simulink model "psm_sv_ekf_bemf_ctrl"  (R2026a)
settings: Solver=ode23tb  StopTime=simlength  FixedStep=tc  MaxStep=tc
values from neighbouring files (symbols this model uses):
  A1_tilde_ekf = [-Rs_norm/Lalpha_norm 0 0 0 0 0; 0 -Rs_norm/Lalpha_norm 0 0 0 0;      0 0 0 0 0 0; 0 0 0 0 0 0;      0 0 0 0 0 1; 0 0 0 0 0 0]    [kalman_psm.m]
  A2_tilde_ekf = [0 0 0 1/Lbeta_norm 0 0; 0 0 -1/Lbeta_norm 0 0 0;      0 0 0 -1 0 0; 0 0 1 0 0 0;     0 0 0 0 0 0; 0 0 0 0 0 0]    [kalman_psm.m]
  A3_tilde_ekf = [0 0 0 0 0 0; 0 0 0 0 0 -1/Lbeta_norm;      0 0 0 0 0 0; 0 0 0 0 0 1;     0 0 0 0 0 0; 0 0 0 0 0 0]    [kalman_psm.m]
  A4_tilde_ekf = [0 0 0 0 0 1/Lalpha_norm; 0 0 0 0 0 0;      0 0 0 0 0 -1; 0 0 0 0 0 0;     0 0 0 0 0 0; 0 0 0 0 0 0]    [kalman_psm.m]
  Bd_ekf = B_tilde_ekf*ts_inv    [kalman_psm.m]
  C_ekf = [1 0 0 0 0 0; 0 1 0 0 0 0]    [kalman_psm.m]
  CTRPIFF_CLIP_RELEASE = 0.001    [init_model.m]
  dead_time_INV = 3e-6    (= 3e-06)    [init_model.m]
  fPWM_INV = fPWM_AFE    (= 5000)    [init_model.m]
  g0_10Hz = fcut_10Hz_flt * ts_afe * 2*pi    (= 0.0125663706144)    [init_model.m]
  g0_1Hz = fcut_1Hz_flt * ts_afe * 2*pi    (= 0.00125663706144)    [init_model.m]
  g1_10Hz = 1 - g0_10Hz    (= 0.987433629386)    [init_model.m]
  g1_1Hz = 1 - g0_1Hz    (= 0.998743362939)    [init_model.m]
  id_lim = 0.35    [init_model.m]
  inv_m_scale = motorc_m_scale    [init_model.m]
  iq_lim = 1.4    [init_model.m]
  kg = Kobs(1)    [init_model.m]
  ki_align = 0.1    [init_model.m]
  ki_i = 18    [init_model.m]
  ki_w = 8    [init_model.m]
  kp_align = 0.6    [init_model.m]
  kp_i = 0.25    [init_model.m]
  kp_w = 2    [init_model.m]
  kw = Kobs(2)    [init_model.m]
  lim_down_align = -0.2    [init_model.m]
  lim_up_align = 0.2    [init_model.m]
  number_of_modules = 1    [init_model.m]
  omega_m_sim = omega_m_bez    [init_model.m]
  Qkalman = ts_inv * [Rs_norm/Lalpha_norm 0 0 0 0 0; 0 Rs_norm/Lbeta_norm 0 0 0 0;      0 0 1 0 0 0;     0 0 0 1 0 0;     0 0 0 0 1 0;     0 0 0 0 0 1]    [kalman_psm.m]
  Rkalman = [ts_inv 0; 0 ts_inv]    [kalman_psm.m]
  simlength = 2    [init_model.m]
  tc = ts_afe/100    (= 2e-06)    [init_model.m]
  time_gain_afe_module_1 = 1.0    (= 1)    [init_model.m]
  time_gain_inv_module_2 = 1.0    (= 1)    [init_model.m]
  time_start_motor_control = 0.025    [init_model.m]
  ts_inv = 1/fPWM_INV    (= 0.0002)    [init_model.m]
undefined symbols (not defined in the file or in its folder): ibez, La, Lb, Ld_norm, Lq_norm, magnitude, omega_bez, omega_m_bez, psi_bez, psi_m, rpm_base, rpm_bez, Rs, tau_bez, torque_base, ubez
libraries: fl_lib x24, nesl_utility x11, cstblocks_lti x2, single_phase_pwm_modulator x1, threephase_inductor_lib x1, simple_flexible_shaft x1, permanent_magnet_synchronous_machine x1
(part 1 of 2)
settings Model: SimulationMode=accelerator  Creator=dbagn  LastModifiedBy=ltnbda
settings SolverCC: NumberNewtonIterations=3.0  ZeroCrossControl=DisableAll  SolverResetMethod=Robust
settings SFSimCC: CustomCodeUndefinedFunction=ThrowError  DefaultCustomCodeDeterministicFunctions=All
settings SFSimCC: SimCustomHeaderCode=|
  | #include "rpi.h"
  | #include "mavgflt.h"
  | #include "mavgflt_simulink.h"
  | #include "mavgflts.h"
  | #include "mavgflts_simulink.h"
  | #include "dsmavgflt.h"
  | #include "dsmavgflt_simulink.h"
  | #include "bemf_obsv.h"
  | #include "bemf_obsv_simulink.h"
  | #include "bemf_obsv_load_est.h"
  | #include "bemf_obsv_load_est_simulink.h"
  | #include "dqvector_pi.h"
  | #include "dqvector_pi_simulink.h"
  | #include "sv_pwm_simulink.h"
  | #include "sv_pwm.h"
  | #include "first_harmonic_tracker.h"
  | #include "first_harmonic_tracker_simulink.h"
  | #include "dqpll_thyr.h"
  | #include "dqpll_thyr_simulink.h"
  | #include "dqpll_grid.h"
  | #include "dqpll_grid_simulink.h"
settings SFSimCC: SimUserSources=|
  | "rpi.c"
  | "mavgflt_simulink.c"
  | "mavgflt.c"
  | "mavgflts_simulink.c"
  | "mavgflts.c"
  | "dsmavgflt_simulink.c"
  | "dsmavgflt.c"
  | "bemf_obsv_simulink.c"
  | "bemf_obsv.c"
  | "bemf_obsv_load_est_simulink.c"
  | "bemf_obsv_load_est.c"
  | "dqvector_pi.c"
  | "dqvector_pi_simulink.c"
  | "sv_pwm_simulink.c"
  | "sv_pwm.c"
  | "first_harmonic_tracker_simulink.c"
  | "first_harmonic_tracker.c"
  | "dqpll_thyr_simulink.c"
  | "dqpll_thyr.c"
  | "dqpll_grid_simulink.c"
  | "dqpll_grid.c"
settings SFSimCC: SimUserIncludeDirs=|
  | include
  | src
settings SimscapeCC: SimscapeNominalValues="[{\"value\":\"1\",\"unit\":\"A\"},{\"value\":\"1\",\"unit\":\"bar\"},{\"value\":\"1\",\"unit\":\"cm^2\"},{\"value\":\"1\",\"unit\":\"cm^3/s\"},{\"value\":\"1\",\"unit\":\"kJ/kg\"},{\"value\":\"1\",\"unit\":\"kW\"},{\"value\":\"1\",\"unit\":\"l\"},{\"value\":\"1\",\"unit\":\"N\"},{\"value\":\"1\",\"unit\":\"N*m\"},{\"value\":\"1\",\"unit\":\"V\"}]"  SimscapeLogType=none  SimscapeLogDataHistory=5000.0

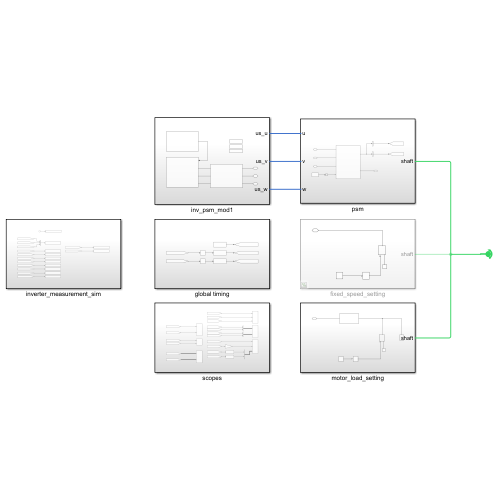
[thumbnail: Simulink's stored preview of the top-level diagram]
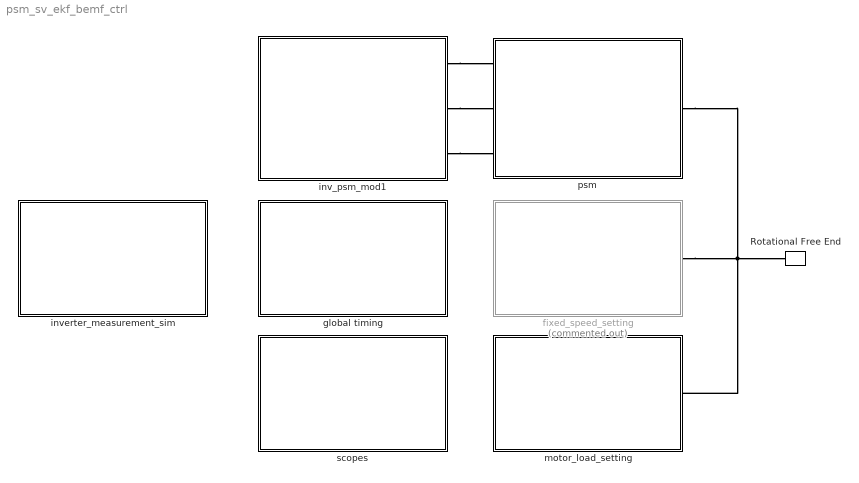
== system psm_sv_ekf_bemf_ctrl ==
  Rotational Free End : fl_lib/Mechanical/Rotational Elements/Rotational Free End  w_specify=off  w_priority=None  w=0 rad/s  w_nominal_specify=off  w_nominal_value=1  w_nominal_unit=rad/s
  fixed_speed_setting : Subsystem  Commented=on
  global timing : Subsystem
  inv_psm_mod1 : Subsystem
  inverter_measurement_sim : Subsystem
  motor_load_setting : Subsystem
  psm : Subsystem
  scopes : Subsystem
  connections:
  psm/RConn1 -- Rotational Free End/LConn1 -- motor_load_setting/LConn1 -- fixed_speed_setting/LConn1
  inv_psm_mod1/RConn2 -- psm/LConn2
  inv_psm_mod1/RConn1 -- psm/LConn1
  inv_psm_mod1/RConn3 -- psm/LConn3

== system psm_sv_ekf_bemf_ctrl/fixed_speed_setting ==
  Ideal Angular Velocity Source : fl_lib/Mechanical/Mechanical Sources/Ideal Angular Velocity Source
  Mechanical Rotational Reference : fl_lib/Mechanical/Rotational Elements/Mechanical Rotational Reference
  PS Step1 : fl_lib/Physical Signals/Sources/PS Step  step_time=0.025 s  initial_value=0 rpm  final_value=rpm_sim rpm
  PS Transfer Function : fl_lib/Physical Signals/Linear Operators/PS Transfer Function  transfer_function_type=foundation.enum.transfer_function_type.lag  T=0.1 s  T1=2 s  T2=1 s  reset_method=foundation.enum.IntegratorResetSpec.None  initial_condition_spec=foundation.enum.IntegratorICSpec.Internal  y0=0 rpm
  shaft : PMIOPort  Side=Left
  connections:
  Mechanical Rotational Reference/LConn1 -- Ideal Angular Velocity Source/RConn2
  PS Step1/RConn1 -- PS Transfer Function/LConn1
  PS Transfer Function/RConn1 -- Ideal Angular Velocity Source/RConn1
  Ideal Angular Velocity Source/LConn1 -- shaft/RConn1

== system psm_sv_ekf_bemf_ctrl/global timing ==
  Unit Delay : UnitDelay  SampleTime=tc
  Unit Delay1 : UnitDelay  SampleTime=tc
  time_afe1 : Subsystem  mask{k=time_gain_afe_module_1}
      mask prompts: k "Time Gain"
      mask Display:
      | disp('time-gen');
      | port_label('input', 1, 'crt');
      | port_label('output', 1, 'tout');
  time_afe3 : Subsystem  mask{k=1}
      mask prompts: k "Time Gain"
      mask Display:
      | disp('time-gen');
      | port_label('output', 1, 'tout');
  time_inv1 : Subsystem  mask{k=time_gain_inv_module_2}
      mask prompts: k "Time Gain"
      mask Display:
      | disp('time-gen');
      | port_label('input', 1, 'crt');
      | port_label('output', 1, 'tout');
  tag scope: time_afe_module_1=global, time_inv_module_1=global, time_master=global
  wires:
  time_afe1/1(Out1) -> [time_afe_module_1]
  time_inv1/1(Out1) -> [time_inv_module_1]
  time_afe3/1(Out1) -> [time_master]
  [local_time_corr_afe1] -> Unit Delay/1
  Unit Delay/1 -> time_afe1/1(correction_time)
  [local_time_corr_inv1] -> Unit Delay1/1
  Unit Delay1/1 -> time_inv1/1(correction_time)

== system psm_sv_ekf_bemf_ctrl/inv_psm_mod1 ==
  Goto Tag Visibility : GotoTagVisibility  GotoTag=uu_ctrl
  Goto Tag Visibility1 : GotoTagVisibility  GotoTag=uv_ctrl
  Goto Tag Visibility2 : GotoTagVisibility  GotoTag=uw_ctrl
  inverter : Subsystem
  inverter_ctrl : Subsystem
  inverter_output_filter : Subsystem
  us_u : PMIOPort  Side=Right
  us_v : PMIOPort  Port=2  Side=Right
  us_w : PMIOPort  Port=3  Side=Right
  wires:
  inverter_ctrl/1(ctrl_out) -> inverter/1(ctrl_out)
  connections:
  inverter/LConn2 -- inverter_output_filter/RConn2
  inverter/LConn1 -- inverter_output_filter/RConn1
  inverter/LConn3 -- inverter_output_filter/RConn3
  inverter_output_filter/LConn2 -- us_v/RConn1
  inverter_output_filter/LConn3 -- us_w/RConn1
  inverter_output_filter/LConn1 -- us_u/RConn1

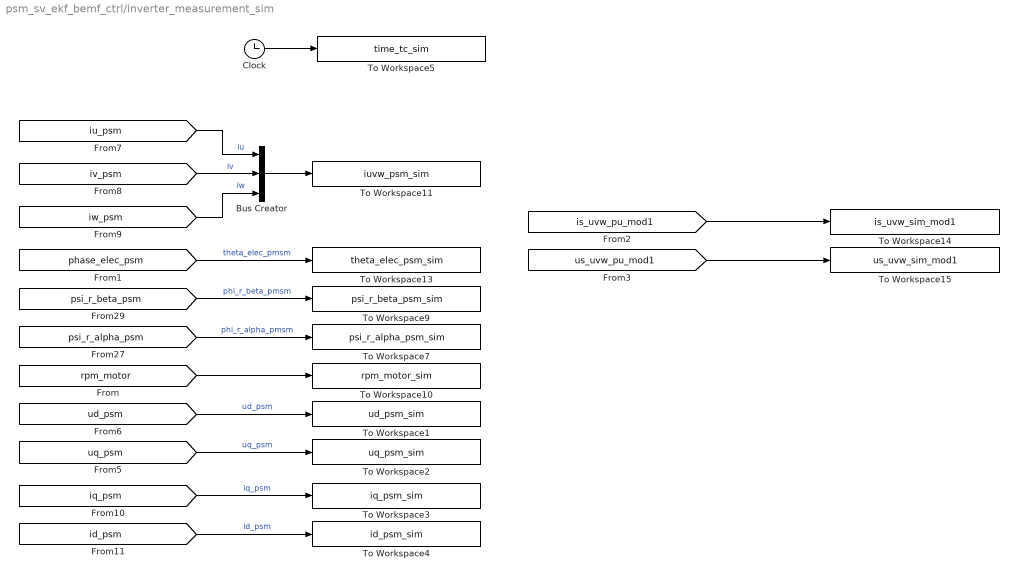
== system psm_sv_ekf_bemf_ctrl/inverter_measurement_sim ==
  Bus Creator : BusCreator  Inputs=3
  Clock : Clock
  To Workspace1 : ToWorkspace  VariableName=ud_psm_sim  SampleTime=tc
      settings: MaxDataPoints=Nc  Save2DSignal=2-D array (concatenate along first dimension)
  To Workspace10 : ToWorkspace  VariableName=rpm_motor_sim  SampleTime=tc
      settings: MaxDataPoints=Nc  Save2DSignal=2-D array (concatenate along first dimension)
  To Workspace11 : ToWorkspace  VariableName=iuvw_psm_sim  SampleTime=tc
      settings: MaxDataPoints=Nc  Save2DSignal=2-D array (concatenate along first dimension)
  To Workspace13 : ToWorkspace  VariableName=theta_elec_psm_sim  SampleTime=tc
      settings: MaxDataPoints=Nc  Save2DSignal=2-D array (concatenate along first dimension)
  To Workspace14 : ToWorkspace  VariableName=is_uvw_sim_mod1  SampleTime=tc
      settings: MaxDataPoints=Nc  Save2DSignal=2-D array (concatenate along first dimension)
  To Workspace15 : ToWorkspace  VariableName=us_uvw_sim_mod1  SampleTime=tc
      settings: MaxDataPoints=Nc  Save2DSignal=2-D array (concatenate along first dimension)
  To Workspace2 : ToWorkspace  VariableName=uq_psm_sim  SampleTime=tc
      settings: MaxDataPoints=Nc  Save2DSignal=2-D array (concatenate along first dimension)
  To Workspace3 : ToWorkspace  VariableName=iq_psm_sim  SampleTime=tc
      settings: MaxDataPoints=Nc  Save2DSignal=2-D array (concatenate along first dimension)
  To Workspace4 : ToWorkspace  VariableName=id_psm_sim  SampleTime=tc
      settings: MaxDataPoints=Nc  Save2DSignal=2-D array (concatenate along first dimension)
  To Workspace5 : ToWorkspace  VariableName=time_tc_sim  SampleTime=tc
      settings: MaxDataPoints=Nc  Save2DSignal=2-D array (concatenate along first dimension)
  To Workspace7 : ToWorkspace  VariableName=psi_r_alpha_psm_sim  SampleTime=tc
      settings: MaxDataPoints=Nc  Save2DSignal=2-D array (concatenate along first dimension)
  To Workspace9 : ToWorkspace  VariableName=psi_r_beta_psm_sim  SampleTime=tc
      settings: MaxDataPoints=Nc  Save2DSignal=2-D array (concatenate along first dimension)
  wires:
  [psi_r_alpha_psm] -> To Workspace7/1  "phi_r_alpha_pmsm"
  [psi_r_beta_psm] -> To Workspace9/1  "phi_r_beta_pmsm"
  [rpm_motor] -> To Workspace10/1
  [iv_psm] -> Bus Creator/2  "iv"
  [iw_psm] -> Bus Creator/3  "iw"
  [iu_psm] -> Bus Creator/1  "iu"
  Bus Creator/1 -> To Workspace11/1
  [phase_elec_psm] -> To Workspace13/1  "theta_elec_pmsm"
  [ud_psm] -> To Workspace1/1  "ud_psm"
  [uq_psm] -> To Workspace2/1  "uq_psm"
  [iq_psm] -> To Workspace3/1  "iq_psm"
  [id_psm] -> To Workspace4/1  "id_psm"
  Clock/1 -> To Workspace5/1
  [is_uvw_pu_mod1] -> To Workspace14/1
  [us_uvw_pu_mod1] -> To Workspace15/1

== system psm_sv_ekf_bemf_ctrl/motor_load_setting ==
  Ideal Torque Source : fl_lib/Mechanical/Mechanical Sources/Ideal Torque Source
  Inertia : fl_lib/Mechanical/Rotational Elements/Inertia  inertia=external_motor_inertia kg*m^2  num_ports=foundation.enum.numPorts2.one  w_specify=off  w_priority=High  w=0 rad/s  w_nominal_specify=off  w_nominal_value=1  w_nominal_unit=rad/s  t_specify=off  t_priority=None  t=0 N*m  t_nominal_specify=off  t_nominal_value=1  t_nominal_unit=N*m
  Mechanical Rotational Reference : fl_lib/Mechanical/Rotational Elements/Mechanical Rotational Reference
  PS Step : fl_lib/Physical Signals/Sources/PS Step  step_time=load_step_time s  initial_value=1 N*m  final_value=1 N*m
  PS Transfer Function : fl_lib/Physical Signals/Linear Operators/PS Transfer Function  transfer_function_type=foundation.enum.transfer_function_type.lag  T=1 s  T1=2 s  T2=1 s  reset_method=foundation.enum.IntegratorResetSpec.None  initial_condition_spec=foundation.enum.IntegratorICSpec.Internal  y0=0 N*m
  flexible_shaft : simple_flexible_shaft/flexible_shaft  b1=1  b2=1  J1=1  J2=1  b_displacement=1  k_displacement=1e5
  shaft : PMIOPort  Side=Left
  connections:
  flexible_shaft/LConn1 -- shaft/RConn1
  Ideal Torque Source/RConn2 -- Mechanical Rotational Reference/LConn1
  PS Transfer Function/RConn1 -- Ideal Torque Source/RConn1
  PS Step/RConn1 -- PS Transfer Function/LConn1
  Ideal Torque Source/LConn1 -- flexible_shaft/RConn1 -- Inertia/LConn1

== system psm_sv_ekf_bemf_ctrl/psm ==
  Bus Selector1 : BusSelector  OutputSignals=omega_mech (rpm)
  Bus Selector2 : BusSelector  OutputSignals=psi_r_alpha (Vs),psi_r_beta (Vs),omega_elec (rad/s),phase_elec (rad)  OutputAsBus=on
  Constant : Constant  Value=psi_m
  Simulink-PS Converter3 : nesl_utility/Simulink-PS Converter  PhysicalDomain=network_engine_domain  SubClassName=ps_input  LeftPortType=input  RightPortType=output  PseudoPeriodic=off  Frequencies=[]  NoiseDistribution=none  NoiseParameters=[]  Unit=V*s  AffineConversion=on  FilteringAndDerivatives=provide  SimscapeFilterOrder=1  InputFilterTimeConstant=0.001  UdotUserProvided=0
  synchronous_motor : Subsystem
  u : PMIOPort  Side=Left
  v : PMIOPort  Port=2  Side=Left
  w : PMIOPort  Port=3  Side=Left
  shaft : PMIOPort  Port=4  Side=Right
  tag scope: motor_fluxes_data=global, rpm_motor=global
  wires:
  synchronous_motor/1(motor_data) -> Bus Selector2/1, Bus Selector1/1
  Bus Selector1/1 -> [rpm_motor]  "<omega_mech (rpm)>"
  Constant/1 -> Simulink-PS Converter3/1
  Bus Selector2/1 -> [motor_fluxes_data]
  connections:
  synchronous_motor/LConn1 -- u/RConn1
  Simulink-PS Converter3/RConn1 -- synchronous_motor/LConn4
  synchronous_motor/LConn3 -- w/RConn1
  synchronous_motor/LConn2 -- v/RConn1
  shaft/RConn1 -- synchronous_motor/RConn1

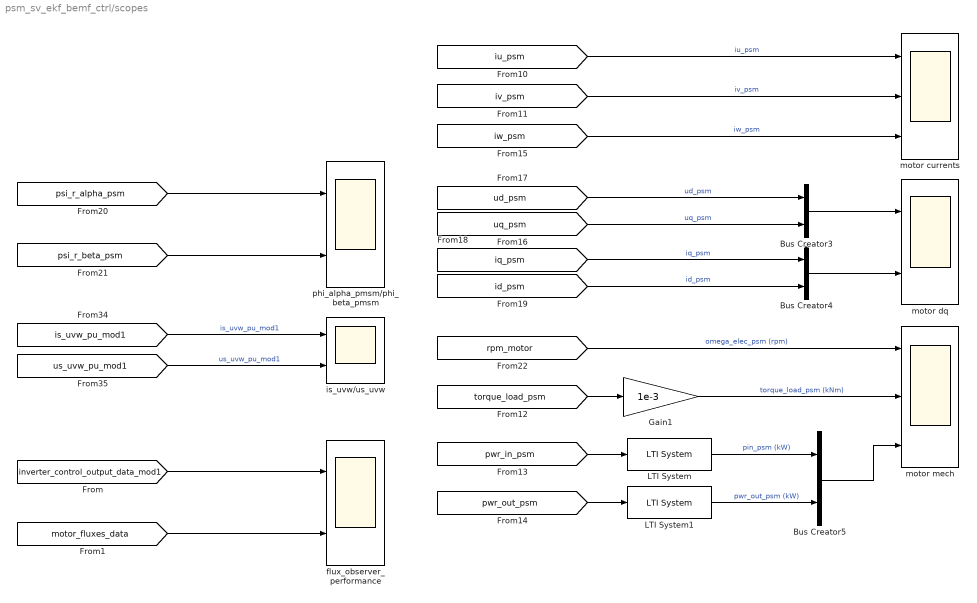
== system psm_sv_ekf_bemf_ctrl/scopes ==
  Bus Creator3 : BusCreator  Inputs=2
  Bus Creator4 : BusCreator  Inputs=2
  Bus Creator5 : BusCreator  Inputs=2
  Gain1 : Gain  Gain=1e-3
  LTI System : cstblocks_lti/LTI System  sys=LVRT_flt_ss_c  IC=[]  PadeOrder=0
  LTI System1 : cstblocks_lti/LTI System  sys=LVRT_flt_ss_c  IC=[]  PadeOrder=0
  flux_observer_performance : Scope  NumInputPorts=2
      settings: SampleTime=tc  ActiveDisplayYMinimum=-0.90724815641806988  ActiveDisplayYMaximum=1.279172141196135
  is_uvw/us_uvw : Scope  NumInputPorts=2
      settings: SampleTime=tc  ActiveDisplayYMinimum=-4.0901889520524559  ActiveDisplayYMaximum=4.1379165768312332  DataLoggingVariableName=ScopeData25
  motor currents : Scope  NumInputPorts=3
      settings: SampleTime=tc  ActiveDisplayYMinimum=-1080.1898447978588  ActiveDisplayYMaximum=1044.7219668898681  DataLoggingVariableName=ScopeData17
  motor dq : Scope  NumInputPorts=2
      settings: SampleTime=tc  ActiveDisplayYMinimum=-581.89506711994022  ActiveDisplayYMaximum=671.86127351087941  DataLoggingVariableName=ScopeData18
  motor mech : Scope  NumInputPorts=3
      settings: SampleTime=tc  ActiveDisplayYMinimum=-2.2245484478220683  ActiveDisplayYMaximum=20.020987845014481  DataLoggingVariableName=ScopeData11
  phi_alpha_pmsm/phi_beta_pmsm : Scope  NumInputPorts=2
      settings: SampleTime=tc  ActiveDisplayYMinimum=-4.8008222938786522  ActiveDisplayYMaximum=4.8008455771888636  DataLoggingVariableName=ScopeData19
  wires:
  [torque_load_psm] -> Gain1/1
  [pwr_out_psm] -> LTI System1/1
  Bus Creator4/1 -> motor dq/2
  LTI System/1 -> Bus Creator5/1  "pin_psm (kW)"
  LTI System1/1 -> Bus Creator5/2  "pwr_out_psm (kW)"
  [iw_psm] -> motor currents/3  "iw_psm"
  Gain1/1 -> motor mech/2  "torque_load_psm (kNm)"
  [id_psm] -> Bus Creator4/2  "id_psm"
  [psi_r_alpha_psm] -> phi_alpha_pmsm/phi_beta_pmsm/1
  [iv_psm] -> motor currents/2  "iv_psm"
  Bus Creator3/1 -> motor dq/1
  [uq_psm] -> Bus Creator3/2  "uq_psm"
  [iu_psm] -> motor currents/1  "iu_psm"
  Bus Creator5/1 -> motor mech/3
  [ud_psm] -> Bus Creator3/1  "ud_psm"
  [iq_psm] -> Bus Creator4/1  "iq_psm"
  [rpm_motor] -> motor mech/1  "omega_elec_psm (rpm)"
  [pwr_in_psm] -> LTI System/1
  [psi_r_beta_psm] -> phi_alpha_pmsm/phi_beta_pmsm/2
  [is_uvw_pu_mod1] -> is_uvw/us_uvw/1  "is_uvw_pu_mod1"
  [us_uvw_pu_mod1] -> is_uvw/us_uvw/2  "us_uvw_pu_mod1"
  [inverter_control_output_data_mod1] -> flux_observer_performance/1
  [motor_fluxes_data] -> flux_observer_performance/2

== system psm_sv_ekf_bemf_ctrl/global timing/time_afe1 ==
  correction_time : Inport
  Constant : Constant
  Gain : Gain  Gain=k
  Product : Product
  Sum : Sum  Inputs=|++
  time_1 : Clock
  Out1 : Outport
  wires:
  time_1/1 -> Gain/1
  Gain/1 -> Product/1
  Product/1 -> Out1/1
  correction_time/1 -> Sum/1
  Sum/1 -> Product/2
  Constant/1 -> Sum/2

== system psm_sv_ekf_bemf_ctrl/global timing/time_afe3 ==
  Gain : Gain  Gain=k
  time_1 : Clock
  Out1 : Outport
  wires:
  Gain/1 -> Out1/1
  time_1/1 -> Gain/1

== system psm_sv_ekf_bemf_ctrl/global timing/time_inv1 ==
  correction_time : Inport
  Constant : Constant
  Gain : Gain  Gain=k
  Product : Product
  Sum : Sum  Inputs=|++
  time_1 : Clock
  Out1 : Outport
  wires:
  time_1/1 -> Gain/1
  Gain/1 -> Product/1
  Product/1 -> Out1/1
  correction_time/1 -> Sum/1
  Constant/1 -> Sum/2
  Sum/1 -> Product/2

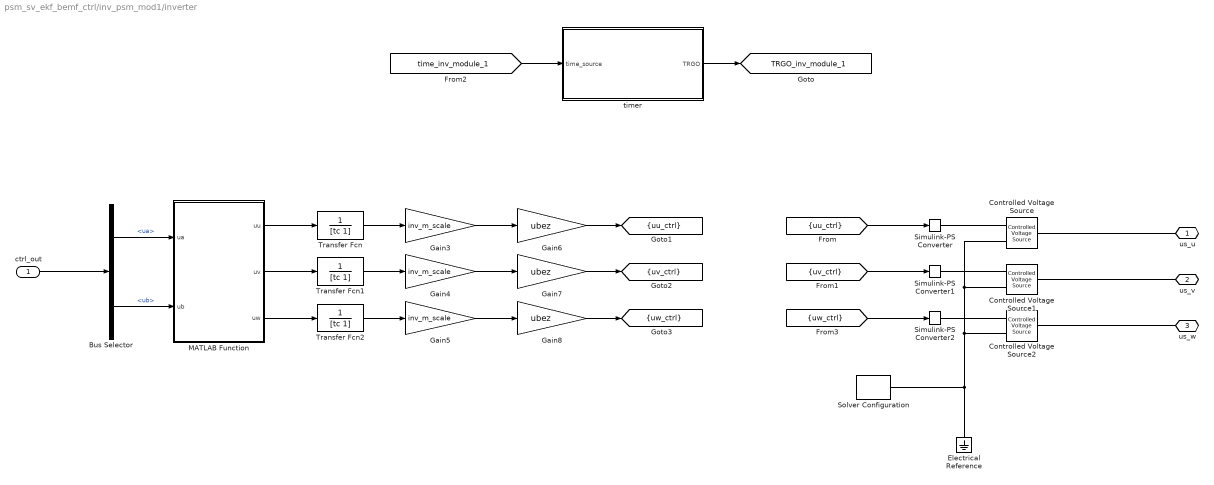
== system psm_sv_ekf_bemf_ctrl/inv_psm_mod1/inverter ==
  ctrl_out : Inport
  Bus Selector : BusSelector  OutputSignals=ua,ub
  Controlled Voltage Source : fl_lib/Electrical/Electrical Sources/Controlled Voltage Source
  Controlled Voltage Source1 : fl_lib/Electrical/Electrical Sources/Controlled Voltage Source
  Controlled Voltage Source2 : fl_lib/Electrical/Electrical Sources/Controlled Voltage Source
  Electrical Reference : fl_lib/Electrical/Electrical Elements/Electrical Reference
  Gain3 : Gain  Gain=inv_m_scale
  Gain4 : Gain  Gain=inv_m_scale
  Gain5 : Gain  Gain=inv_m_scale
  Gain6 : Gain  Gain=ubez
  Gain7 : Gain  Gain=ubez
  Gain8 : Gain  Gain=ubez
  MATLAB Function : MATLAB Function  TreatAsAtomicUnit=on
  Simulink-PS Converter : nesl_utility/Simulink-PS Converter  PhysicalDomain=network_engine_domain  SubClassName=ps_input  LeftPortType=input  RightPortType=output  PseudoPeriodic=off  Frequencies=[]  NoiseDistribution=none  NoiseParameters=[]  Unit=V  AffineConversion=off  FilteringAndDerivatives=provide  SimscapeFilterOrder=1  InputFilterTimeConstant=0.001  UdotUserProvided=0
  Simulink-PS Converter1 : nesl_utility/Simulink-PS Converter  PhysicalDomain=network_engine_domain  SubClassName=ps_input  LeftPortType=input  RightPortType=output  PseudoPeriodic=off  Frequencies=[]  NoiseDistribution=none  NoiseParameters=[]  Unit=V  AffineConversion=off  FilteringAndDerivatives=provide  SimscapeFilterOrder=1  InputFilterTimeConstant=0.001  UdotUserProvided=0
  Simulink-PS Converter2 : nesl_utility/Simulink-PS Converter  PhysicalDomain=network_engine_domain  SubClassName=ps_input  LeftPortType=input  RightPortType=output  PseudoPeriodic=off  Frequencies=[]  NoiseDistribution=none  NoiseParameters=[]  Unit=V  AffineConversion=off  FilteringAndDerivatives=provide  SimscapeFilterOrder=1  InputFilterTimeConstant=0.001  UdotUserProvided=0
  Solver Configuration : nesl_utility/Solver Configuration  PhysicalDomain=network_engine_domain  SubClassName=solver  LeftPortType=input  RightPortType=generic  Tones=[]  Harmonics=[]  SimulateNoise=off  Profile=off  UseLocalSampling=off  EnableSwitchedLinearOptims=on  FrequencyDomain=off  UseCCode=off  RelTol=0.001  AbsTol=0.001  MinStep=1e-09  ToWorkspace=off  RevertToSquareIcSolve=off  NumHomotopyIterations=100  PhasorMode=off  PhasorModeNumHarmonics=1  ConsistencySolver=NEWTON_XTOL_AFTER_FTOL  CanonicalOrdering=UNORDERED  OptimizeIntermediates=UNOPTIMIZED  IndexReductionMethod=DerivativeReplacement  DoDC=off  ResidualTolerance=1e-09  ConsistencyTolSource=GLOBAL  ConsistencyAbsTol=0.001  ConsistencyRelTol=0.001  ConsistencyTolFactor=0.001  UseLocalSolver=on  LocalSolverChoice=NE_BACKWARD_EULER_ADVANCER  ResolveIndetEquations=on  FunctionEvalNumThread=1  LocalSolverSampleTime=tc  DoFixedCost=on  MaxNonlinIter=3  MaxModeIter=2  ComputeImpulses=off  ImpulseIterations=2  LinearAlgebra=auto  LinearAlgebraNumThread=0  EquationFormulation=NE_TIME_EF  DelaysMemoryBudget=1024  AutomaticFiltering=on  FilteringTimeConstant=0.001  PartitionStorageMethod=AS_NEEDED  PartitionMemoryBudget=1024  PartitionMethod=ROBUST  MultibodyUseLocalSolver=off  MultibodyLocalSolverChoice=ODE1  MultibodyLocalSolverSampleTime=0.001
  Transfer Fcn : TransferFcn  Denominator=[tc 1]
  Transfer Fcn1 : TransferFcn  Denominator=[tc 1]
  Transfer Fcn2 : TransferFcn  Denominator=[tc 1]
  timer : Subsystem  mask{f=fPWM_INV, m_up=0.98, m_low=0.02, dead_time=dead_time_INV, pos_cmd_gate=15, neg_cmd_gate=-10, polarity=1, tc=tc, double_sampling=0}
      mask prompts: f "Frequency (Hz)"; m_up "Max Input Modulation Value"; m_low "Min Input Modulation Value"; dead_time "Dead Time (s)"; pos_cmd_gate "Positive Gate Voltage (V)"; neg_cmd_gate "Negative Gate Voltage (V)"; polarity "Polarity (pu)"; tc "Sampling time"
  us_u : PMIOPort  Side=Left
  us_v : PMIOPort  Port=2  Side=Left
  us_w : PMIOPort  Port=3  Side=Left
  tag scope: TRGO_inv_module_1=global, uu_ctrl=scoped, uv_ctrl=scoped, uw_ctrl=scoped
  wires:
  [time_inv_module_1] -> timer/1(time_source)
  timer/1(TRGO) -> [TRGO_inv_module_1]
  ctrl_out/1 -> Bus Selector/1
  Bus Selector/1 -> MATLAB Function/1(ua)  "<ua>"
  Bus Selector/2 -> MATLAB Function/2(ub)  "<ub>"
  MATLAB Function/1(uu) -> Transfer Fcn/1
  MATLAB Function/2(uv) -> Transfer Fcn1/1
  MATLAB Function/3(uw) -> Transfer Fcn2/1
  [uu_ctrl] -> Simulink-PS Converter/1
  [uv_ctrl] -> Simulink-PS Converter1/1
  [uw_ctrl] -> Simulink-PS Converter2/1
  Transfer Fcn/1 -> Gain3/1
  Transfer Fcn1/1 -> Gain4/1
  Transfer Fcn2/1 -> Gain5/1
  Gain4/1 -> Gain7/1
  Gain5/1 -> Gain8/1
  Gain3/1 -> Gain6/1
  Gain6/1 -> [uu_ctrl]
  Gain7/1 -> [uv_ctrl]
  Gain8/1 -> [uw_ctrl]
  connections:
  Controlled Voltage Source/LConn1 -- us_u/RConn1
  Controlled Voltage Source1/LConn1 -- us_v/RConn1
  Controlled Voltage Source2/LConn1 -- us_w/RConn1
  Simulink-PS Converter/RConn1 -- Controlled Voltage Source/RConn1
  Simulink-PS Converter1/RConn1 -- Controlled Voltage Source1/RConn1
  Simulink-PS Converter2/RConn1 -- Controlled Voltage Source2/RConn1
  Electrical Reference/LConn1 -- Solver Configuration/RConn1 -- Controlled Voltage Source2/RConn2 -- Controlled Voltage Source1/RConn2 -- Controlled Voltage Source/RConn2

== system psm_sv_ekf_bemf_ctrl/inv_psm_mod1/inverter_ctrl ==
  Constant : Constant
  inverter_control : Subsystem
  ctrl_out : Outport
  tag scope: inverter_control_output_data_mod1=global, local_time_corr_inv1=global, master_torque_ref=global
  wires:
  [is_uvw_pu_mod1] -> inverter_control/1(is_uvw)
  [TRGO_inv_module_1] -> inverter_control/Trigger
  Constant/1 -> inverter_control/2(udc_pu)
  inverter_control/1(ctrl_out) -> ctrl_out/1
  [time_inv_module_1] -> inverter_control/3(local_time)
  [time_master] -> inverter_control/4(master_time)
  inverter_control/2(local_time_corr) -> [local_time_corr_inv1]
  inverter_control/3(master_torque_ref) -> [master_torque_ref]
  [phase_elec_psm] -> inverter_control/5(phase_elec_psm)
  [omega_elec_psm] -> inverter_control/6(omega_elec_psm)
  inverter_control/4(output_data) -> [inverter_control_output_data_mod1]

== system psm_sv_ekf_bemf_ctrl/inv_psm_mod1/inverter_output_filter ==
  Inductor : fl_lib/Electrical/Electrical Elements/Inductor  l=1e-6 H  r=0 Ohm  g=1e-9 1/Ohm  i_specify=off  i_priority=None  i=0 A  i_nominal_specify=off  i_nominal_value=1  i_nominal_unit=A  v_specify=off  v_priority=None  v=0 V  v_nominal_specify=off  v_nominal_value=1  v_nominal_unit=V  i_L_specify=off  i_L_priority=High  i_L=0 A  i_L_nominal_specify=off  i_L_nominal_value=1  i_L_nominal_unit=A
  Inductor1 : fl_lib/Electrical/Electrical Elements/Inductor  l=1e-6 H  r=0 Ohm  g=1e-9 1/Ohm  i_specify=off  i_priority=None  i=0 A  i_nominal_specify=off  i_nominal_value=1  i_nominal_unit=A  v_specify=off  v_priority=None  v=0 V  v_nominal_specify=off  v_nominal_value=1  v_nominal_unit=V  i_L_specify=off  i_L_priority=High  i_L=0 A  i_L_nominal_specify=off  i_L_nominal_value=1  i_L_nominal_unit=A
  Inductor2 : fl_lib/Electrical/Electrical Elements/Inductor  l=1e-6 H  r=0 Ohm  g=1e-9 1/Ohm  i_specify=off  i_priority=None  i=0 A  i_nominal_specify=off  i_nominal_value=1  i_nominal_unit=A  v_specify=off  v_priority=None  v=0 V  v_nominal_specify=off  v_nominal_value=1  v_nominal_unit=V  i_L_specify=off  i_L_priority=High  i_L=0 A  i_L_nominal_specify=off  i_L_nominal_value=1  i_L_nominal_unit=A
  threephase inductor : threephase_inductor_lib/threephase inductor  Lp=LFi H  L0=LFi_0 H  Rp=2.4e-3 Ohm  R0=0.8e-3 Ohm  Lls=5e-6 H  uu_1_specify=off  uu_1_priority=None  uu_1=0 V  uu_1_nominal_specify=off  uu_1_nominal_value=1  uu_1_nominal_unit=V  uv_1_specify=off  uv_1_priority=None  uv_1=0 V  uv_1_nominal_specify=off  uv_1_nominal_value=1  uv_1_nominal_unit=V  uw_1_specify=off  uw_1_priority=None  uw_1=0 V  uw_1_nominal_specify=off  uw_1_nominal_value=1  uw_1_nominal_unit=V  uu_2_specify=off  uu_2_priority=None  uu_2=0 V  uu_2_nominal_specify=off  uu_2_nominal_value=1  uu_2_nominal_unit=V  uv_2_specify=off  uv_2_priority=None  uv_2=0 V  uv_2_nominal_specify=off  uv_2_nominal_value=1  uv_2_nominal_unit=V  uw_2_specify=off  uw_2_priority=None  uw_2=0 V  uw_2_nominal_specify=off  uw_2_nominal_value=1  uw_2_nominal_unit=V  iu_specify=off  iu_priority=None  iu=0 A  iu_nominal_specify=off  iu_nominal_value=1  iu_nominal_unit=A  iv_specify=off  iv_priority=None  iv=0 A  iv_nominal_specify=off  iv_nominal_value=1  iv_nominal_unit=A  iw_specify=off  iw_priority=None  iw=0 A  iw_nominal_specify=off  iw_nominal_value=1  iw_nominal_unit=A
  threephase_vi_measures_stack : Subsystem
  us_u : PMIOPort  Side=Left
  uu : PMIOPort  Port=2  Side=Right
  us_v : PMIOPort  Port=3  Side=Left
  uv : PMIOPort  Port=4  Side=Right
  us_w : PMIOPort  Port=5  Side=Left
  uw : PMIOPort  Port=6  Side=Right
  connections:
  threephase_vi_measures_stack/LConn1 -- us_u/RConn1
  threephase_vi_measures_stack/LConn2 -- us_v/RConn1
  threephase_vi_measures_stack/LConn3 -- us_w/RConn1
  threephase inductor/LConn1 -- threephase_vi_measures_stack/RConn1
  threephase inductor/LConn2 -- threephase_vi_measures_stack/RConn2
  threephase inductor/LConn3 -- threephase_vi_measures_stack/RConn3
  threephase inductor/RConn1 -- Inductor/LConn1
  threephase inductor/RConn2 -- Inductor1/LConn1
  threephase inductor/RConn3 -- Inductor2/LConn1
  Inductor/RConn1 -- uu/RConn1
  Inductor1/RConn1 -- uv/RConn1
  Inductor2/RConn1 -- uw/RConn1

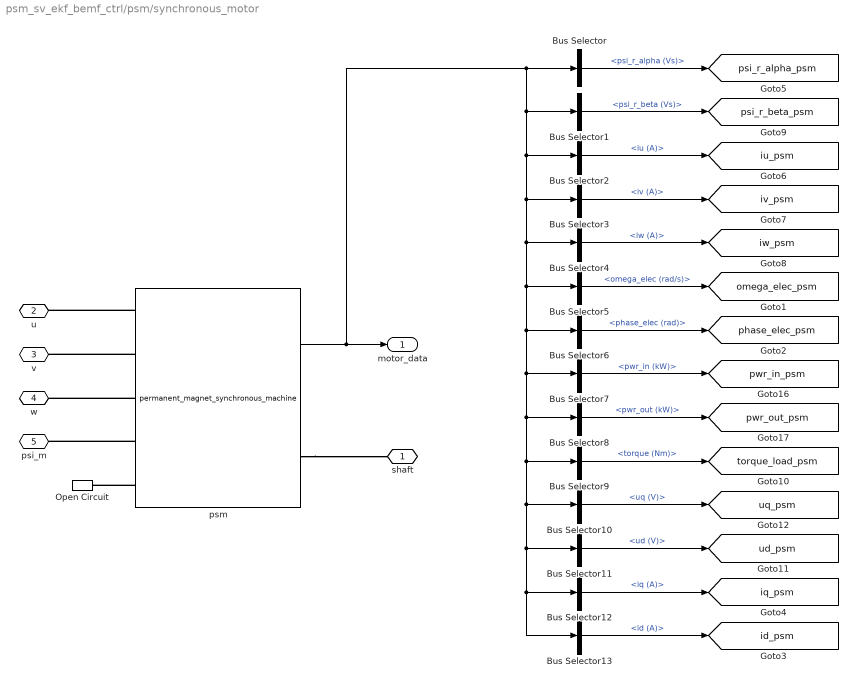
== system psm_sv_ekf_bemf_ctrl/psm/synchronous_motor ==
  Bus Selector : BusSelector  OutputSignals=psi_r_alpha (Vs)
  Bus Selector1 : BusSelector  OutputSignals=psi_r_beta (Vs)
  Bus Selector10 : BusSelector  OutputSignals=uq (V)
  Bus Selector11 : BusSelector  OutputSignals=ud (V)
  Bus Selector12 : BusSelector  OutputSignals=iq (A)
  Bus Selector13 : BusSelector  OutputSignals=id (A)
  Bus Selector2 : BusSelector  OutputSignals=iu (A)
  Bus Selector3 : BusSelector  OutputSignals=iv (A)
  Bus Selector4 : BusSelector  OutputSignals=iw (A)
  Bus Selector5 : BusSelector  OutputSignals=omega_elec (rad/s)
  Bus Selector6 : BusSelector  OutputSignals=phase_elec (rad)
  Bus Selector7 : BusSelector  OutputSignals=pwr_in (kW)
  Bus Selector8 : BusSelector  OutputSignals=pwr_out (kW)
  Bus Selector9 : BusSelector  OutputSignals=torque (Nm)
  Open Circuit : fl_lib/Electrical/Electrical Elements/Open Circuit  v_specify=off  v_priority=None  v=0 V  v_nominal_specify=off  v_nominal_value=1  v_nominal_unit=V
  psm : permanent_magnet_synchronous_machine/permanent_magnet_synchronous_machine  pp=number_poles  psi_m=psi_m  Lmu=5e-6  La=La/number_of_modules  Lb=Lb/number_of_modules  Rs=Rs/number_of_modules  Jm=Jm  b_linear=b  b_quadratic=0  h5_percent=0  h7_percent=0  psi_r_u_init=psi_m  psi_r_v_init=-psi_m/2  psi_r_w_init=-psi_m/2  omega_init=0  phase_init=0
  shaft : PMIOPort  Side=Right
  u : PMIOPort  Port=2  Side=Left
  v : PMIOPort  Port=3  Side=Left
  w : PMIOPort  Port=4  Side=Left
  psi_m : PMIOPort  Port=5  Side=Left
  motor_data : Outport
  tag scope: id_psm=global, iq_psm=global, iu_psm=global, iv_psm=global, iw_psm=global, omega_elec_psm=global, phase_elec_psm=global, psi_r_alpha_psm=global, psi_r_beta_psm=global, pwr_in_psm=global, pwr_out_psm=global, torque_load_psm=global, ud_psm=global, uq_psm=global
  wires:
  psm/1 -> Bus Selector8/1, Bus Selector10/1, Bus Selector11/1, Bus Selector12/1, Bus Selector13/1, Bus Selector9/1, Bus Selector7/1, Bus Selector6/1, Bus Selector5/1, Bus Selector4/1, Bus Selector3/1, Bus Selector2/1, Bus Selector1/1, Bus Selector/1, motor_data/1
  Bus Selector/1 -> [psi_r_alpha_psm]  "<psi_r_alpha (Vs)>"
  Bus Selector1/1 -> [psi_r_beta_psm]  "<psi_r_beta (Vs)>"
  Bus Selector2/1 -> [iu_psm]  "<iu (A)>"
  Bus Selector3/1 -> [iv_psm]  "<iv (A)>"
  Bus Selector4/1 -> [iw_psm]  "<iw (A)>"
  Bus Selector5/1 -> [omega_elec_psm]  "<omega_elec (rad/s)>"
  Bus Selector6/1 -> [phase_elec_psm]  "<phase_elec (rad)>"
  Bus Selector7/1 -> [pwr_in_psm]  "<pwr_in (kW)>"
  Bus Selector8/1 -> [pwr_out_psm]  "<pwr_out (kW)>"
  Bus Selector9/1 -> [torque_load_psm]  "<torque (Nm)>"
  Bus Selector10/1 -> [uq_psm]  "<uq (V)>"
  Bus Selector11/1 -> [ud_psm]  "<ud (V)>"
  Bus Selector12/1 -> [iq_psm]  "<iq (A)>"
  Bus Selector13/1 -> [id_psm]  "<id (A)>"
  connections:
  psm/RConn1 -- shaft/RConn1
  psm/LConn1 -- u/RConn1
  psm/LConn2 -- v/RConn1
  psm/LConn3 -- w/RConn1
  psm/LConn4 -- psi_m/RConn1
  psm/LConn5 -- Open Circuit/LConn1

== system psm_sv_ekf_bemf_ctrl/inv_psm_mod1/inverter/timer ==
  time_source : Inport
  Constant1 : Constant  Value=double_sampling
  Constant2 : Constant  Value=0
  Constant8 : Constant  Value=tc
  Constant9 : Constant  Value=f
  MATLAB Function : MATLAB Function  TreatAsAtomicUnit=on  SystemSampleTime=tc
  MATLAB Function1 : single_phase_pwm_modulator/Single phase two level PWM generator with global TRGO/MATLAB Function1  SystemSampleTime=tc  VariantActivationTime=update diagram  EmptyChoice=off  PassThrough=off  PassThroughVariantControl=(default)  EmptyChoiceVariantControl=(default)  AllowFlexibleInterface=on  Latency=0  AutoFrameSizeCalculation=off
  period : Constant  Value=1/f
  TRGO : Outport
  wires:
  Constant1/1 -> MATLAB Function1/4
  time_source/1 -> MATLAB Function/1(t)
  Constant9/1 -> MATLAB Function1/2
  Constant8/1 -> MATLAB Function1/1
  MATLAB Function1/1 -> TRGO/1
  MATLAB Function/1(y) -> MATLAB Function1/3
  Constant2/1 -> MATLAB Function/2(phase)
  period/1 -> MATLAB Function/3(period)

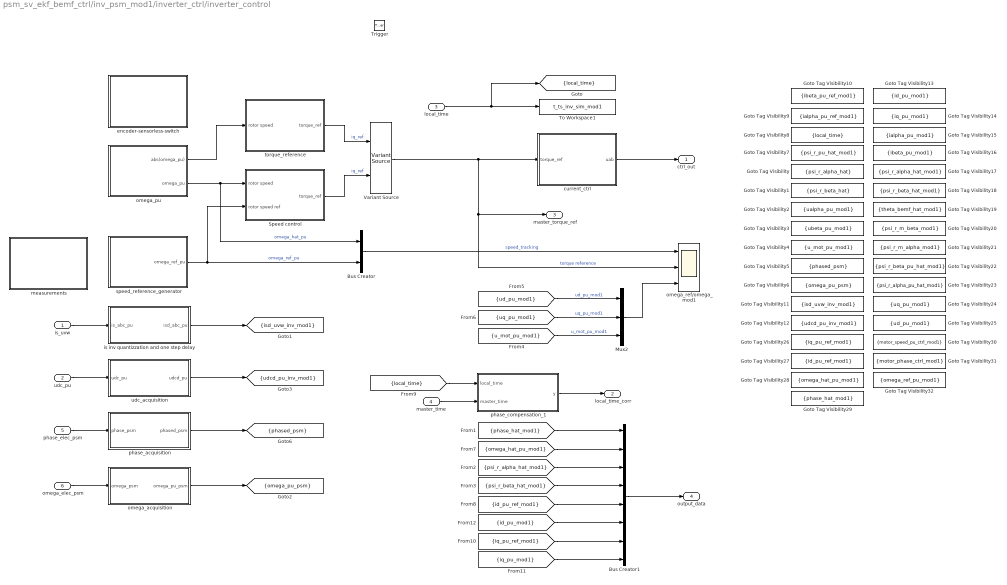
== system psm_sv_ekf_bemf_ctrl/inv_psm_mod1/inverter_ctrl/inverter_control ==
  is_uvw : Inport
  udc_pu : Inport  Port=2
  local_time : Inport  Port=3
  master_time : Inport  Port=4
  phase_elec_psm : Inport  Port=5
  omega_elec_psm : Inport  Port=6
  Trigger : TriggerPort  VariantControl=(inherit)  PortDimensions=1
  Bus Creator : BusCreator  Inputs=2
  Bus Creator1 : BusCreator  Inputs=8
  Goto Tag Visibility : GotoTagVisibility  GotoTag=psi_r_alpha_hat
  Goto Tag Visibility1 : GotoTagVisibility  GotoTag=psi_r_beta_hat
  Goto Tag Visibility10 : GotoTagVisibility  GotoTag=ibeta_pu_ref_mod1
  Goto Tag Visibility11 : GotoTagVisibility  GotoTag=isd_uvw_inv_mod1
  Goto Tag Visibility12 : GotoTagVisibility  GotoTag=udcd_pu_inv_mod1
  Goto Tag Visibility13 : GotoTagVisibility  GotoTag=id_pu_mod1
  Goto Tag Visibility14 : GotoTagVisibility  GotoTag=iq_pu_mod1
  Goto Tag Visibility15 : GotoTagVisibility  GotoTag=ialpha_pu_mod1
  Goto Tag Visibility16 : GotoTagVisibility  GotoTag=ibeta_pu_mod1
  Goto Tag Visibility17 : GotoTagVisibility  GotoTag=psi_r_alpha_hat_mod1
  Goto Tag Visibility18 : GotoTagVisibility  GotoTag=psi_r_beta_hat_mod1
  Goto Tag Visibility19 : GotoTagVisibility  GotoTag=theta_bemf_hat_mod1
  Goto Tag Visibility2 : GotoTagVisibility  GotoTag=ualpha_pu_mod1
  Goto Tag Visibility20 : GotoTagVisibility  GotoTag=psi_r_m_beta_mod1
  Goto Tag Visibility21 : GotoTagVisibility  GotoTag=psi_r_m_alpha_mod1
  Goto Tag Visibility22 : GotoTagVisibility  GotoTag=psi_r_beta_pu_hat_mod1
  Goto Tag Visibility23 : GotoTagVisibility  GotoTag=psi_r_alpha_pu_hat_mod1
  Goto Tag Visibility24 : GotoTagVisibility  GotoTag=uq_pu_mod1
  Goto Tag Visibility25 : GotoTagVisibility  GotoTag=ud_pu_mod1
  Goto Tag Visibility26 : GotoTagVisibility  GotoTag=iq_pu_ref_mod1
  Goto Tag Visibility27 : GotoTagVisibility  GotoTag=id_pu_ref_mod1
  Goto Tag Visibility28 : GotoTagVisibility  GotoTag=omega_hat_pu_mod1
  Goto Tag Visibility29 : GotoTagVisibility  GotoTag=phase_hat_mod1
  Goto Tag Visibility3 : GotoTagVisibility  GotoTag=ubeta_pu_mod1
  Goto Tag Visibility30 : GotoTagVisibility  GotoTag=motor_speed_pu_ctrl_mod1
  Goto Tag Visibility31 : GotoTagVisibility  GotoTag=motor_phase_ctrl_mod1
  Goto Tag Visibility32 : GotoTagVisibility  GotoTag=omega_ref_pu_mod1
  Goto Tag Visibility4 : GotoTagVisibility  GotoTag=u_mot_pu_mod1
  Goto Tag Visibility5 : GotoTagVisibility  GotoTag=phased_psm
  Goto Tag Visibility6 : GotoTagVisibility  GotoTag=omega_pu_psm
  Goto Tag Visibility7 : GotoTagVisibility  GotoTag=psi_r_pu_hat_mod1
  Goto Tag Visibility8 : GotoTagVisibility  GotoTag=local_time
  Goto Tag Visibility9 : GotoTagVisibility  GotoTag=ialpha_pu_ref_mod1
  Mux2 : Mux  Inputs=3
  Speed control : Subsystem
  To Workspace1 : ToWorkspace  VariableName=t_ts_inv_sim_mod1  SampleTime=-1
      settings: MaxDataPoints=Ns_afe
  Variant Source : VariantSource  VariantControls={use_torque_curve == 1, use_speed_control == 1}
  current_ctrl : Subsystem
  encoder-sensorless-switch : Subsystem
  is inv quantizzation and one step delay : Subsystem
  measurements : Subsystem
  omega_acquisition : Subsystem
  omega_pu : Subsystem
  omega_ref/omega_mod1 : Scope  NumInputPorts=3
      settings: ActiveDisplayYMinimum=-0.40440601573274715  ActiveDisplayYMaximum=1.1433678819820206  DataLoggingVariableName=ScopeData3
  phase_acquisition : Subsystem
  phase_compensation_1 : Subsystem
  speed_reference_generator : Subsystem
  torque_reference : Subsystem
  udc_acquisition : Subsystem
  ctrl_out : Outport  VectorParamsAs1DForOutWhenUnconnected=off
  local_time_corr : Outport  Port=2
  master_torque_ref : Outport  Port=3  VectorParamsAs1DForOutWhenUnconnected=off
  output_data : Outport  Port=4
  tag scope: isd_uvw_inv_mod1=scoped, local_time=scoped, omega_pu_psm=scoped, phased_psm=scoped, udcd_pu_inv_mod1=scoped
  wires:
  speed_reference_generator/1(omega_ref_pu) -> Speed control/2(rotor speed ref), Bus Creator/2  "omega_ref_pu"
  Bus Creator/1 -> omega_ref/omega_mod1/1  "speed_tracking"
  Variant Source/1 -> current_ctrl/1(torque_ref), master_torque_ref/1, omega_ref/omega_mod1/2  "torque reference"
  [ud_pu_mod1] -> Mux2/1  "ud_pu_mod1"
  [uq_pu_mod1] -> Mux2/2  "uq_pu_mod1"
  Mux2/1 -> omega_ref/omega_mod1/3
  [u_mot_pu_mod1] -> Mux2/3  "u_mot_pu_mod1"
  omega_pu/2(omega_pu) -> Bus Creator/1, Speed control/1(rotor speed)  "omega_hat_pu"
  omega_pu/1(abs(omega_pu)) -> torque_reference/1(rotor speed)
  torque_reference/1(torque_ref) -> Variant Source/1  "iq_ref"
  Speed control/1(torque_ref) -> Variant Source/2  "iq_ref"
  udc_acquisition/1(udcd_pu) -> [udcd_pu_inv_mod1]
  udc_pu/1 -> udc_acquisition/1(udc_pu)
  is_uvw/1 -> is inv quantizzation and one step delay/1(is_abc_pu)
  is inv quantizzation and one step delay/1(isd_abc_pu) -> [isd_uvw_inv_mod1]
  local_time/1 -> To Workspace1/1, [local_time]
  current_ctrl/1(uab) -> ctrl_out/1
  master_time/1 -> phase_compensation_1/2(master_time)
  [local_time] -> phase_compensation_1/1(local_time)
  phase_compensation_1/1(y) -> local_time_corr/1
  phase_acquisition/1(phased_psm) -> [phased_psm]
  phase_elec_psm/1 -> phase_acquisition/1(phase_psm)
  omega_elec_psm/1 -> omega_acquisition/1(omega_psm)
  omega_acquisition/1(omega_pu_psm) -> [omega_pu_psm]
  [phase_hat_mod1] -> Bus Creator1/1
  [omega_hat_pu_mod1] -> Bus Creator1/2
  [psi_r_alpha_hat_mod1] -> Bus Creator1/3
  [psi_r_beta_hat_mod1] -> Bus Creator1/4
  [id_pu_ref_mod1] -> Bus Creator1/5
  [id_pu_mod1] -> Bus Creator1/6
  [iq_pu_ref_mod1] -> Bus Creator1/7
  [iq_pu_mod1] -> Bus Creator1/8
  Bus Creator1/1 -> output_data/1

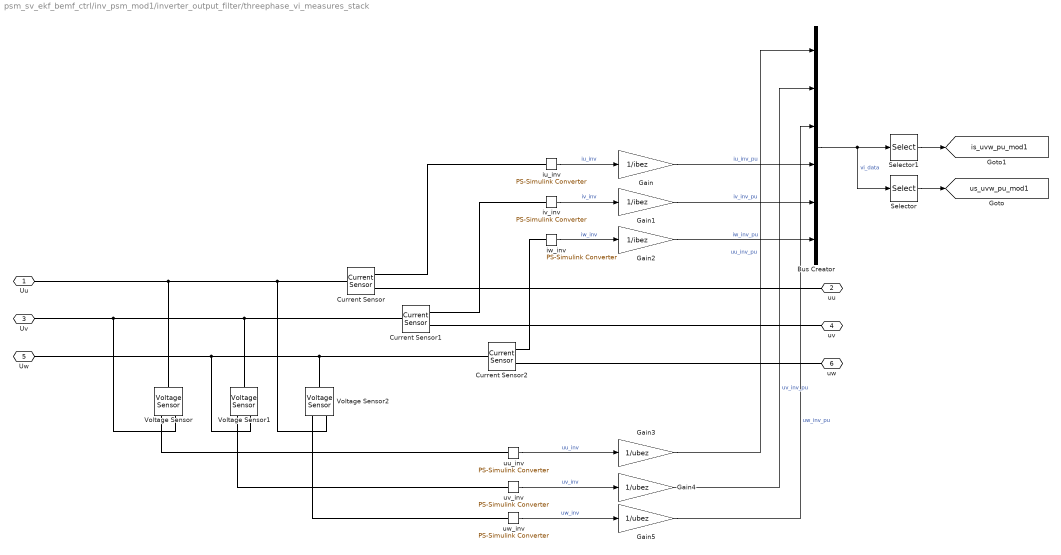
== system psm_sv_ekf_bemf_ctrl/inv_psm_mod1/inverter_output_filter/threephase_vi_measures_stack ==
  Bus Creator : BusCreator  Inputs=6
  Current Sensor : fl_lib/Electrical/Electrical Sensors/Current Sensor
  Current Sensor1 : fl_lib/Electrical/Electrical Sensors/Current Sensor
  Current Sensor2 : fl_lib/Electrical/Electrical Sensors/Current Sensor
  Gain : Gain  Gain=1/ibez
  Gain1 : Gain  Gain=1/ibez
  Gain2 : Gain  Gain=1/ibez
  Gain3 : Gain  Gain=1/ubez
  Gain4 : Gain  Gain=1/ubez
  Gain5 : Gain  Gain=1/ubez
  Selector : Selector  InputPortWidth=6  IndexOptions=Index vector (dialog)  Indices=[1 2 3]  OutputSizes=1
  Selector1 : Selector  InputPortWidth=6  IndexOptions=Index vector (dialog)  Indices=[4 5 6]  OutputSizes=1
  Voltage Sensor : fl_lib/Electrical/Electrical Sensors/Voltage Sensor
  Voltage Sensor1 : fl_lib/Electrical/Electrical Sensors/Voltage Sensor
  Voltage Sensor2 : fl_lib/Electrical/Electrical Sensors/Voltage Sensor
  iu_inv : nesl_utility/PS-Simulink Converter  PhysicalDomain=network_engine_domain  SubClassName=ps_output  LeftPortType=input  RightPortType=output  PseudoPeriodic=off  Frequencies=[]  VectorFormat=1-D array  Unit=A  AffineConversion=off
  iv_inv : nesl_utility/PS-Simulink Converter  PhysicalDomain=network_engine_domain  SubClassName=ps_output  LeftPortType=input  RightPortType=output  PseudoPeriodic=off  Frequencies=[]  VectorFormat=1-D array  Unit=A  AffineConversion=off
  iw_inv : nesl_utility/PS-Simulink Converter  PhysicalDomain=network_engine_domain  SubClassName=ps_output  LeftPortType=input  RightPortType=output  PseudoPeriodic=off  Frequencies=[]  VectorFormat=1-D array  Unit=A  AffineConversion=off
  uu_inv : nesl_utility/PS-Simulink Converter  PhysicalDomain=network_engine_domain  SubClassName=ps_output  LeftPortType=input  RightPortType=output  PseudoPeriodic=off  Frequencies=[]  VectorFormat=1-D array  Unit=V  AffineConversion=off
  uv_inv : nesl_utility/PS-Simulink Converter  PhysicalDomain=network_engine_domain  SubClassName=ps_output  LeftPortType=input  RightPortType=output  PseudoPeriodic=off  Frequencies=[]  VectorFormat=1-D array  Unit=V  AffineConversion=off
  uw_inv : nesl_utility/PS-Simulink Converter  PhysicalDomain=network_engine_domain  SubClassName=ps_output  LeftPortType=input  RightPortType=output  PseudoPeriodic=off  Frequencies=[]  VectorFormat=1-D array  Unit=V  AffineConversion=off
  Uu : PMIOPort  Side=Left
  uu : PMIOPort  Port=2  Side=Right
  Uv : PMIOPort  Port=3  Side=Left
  uv : PMIOPort  Port=4  Side=Right
  Uw : PMIOPort  Port=5  Side=Left
  uw : PMIOPort  Port=6  Side=Right
  tag scope: is_uvw_pu_mod1=global, us_uvw_pu_mod1=global
  wires:
  Bus Creator/1 -> Selector/1, Selector1/1  "vi_data"
  Selector/1 -> [us_uvw_pu_mod1]
  iv_inv/1 -> Gain1/1  "iv_inv"
  iu_inv/1 -> Gain/1  "iu_inv"
  iw_inv/1 -> Gain2/1  "iw_inv"
  uu_inv/1 -> Gain3/1  "uu_inv"
  uv_inv/1 -> Gain4/1  "uv_inv"
  uw_inv/1 -> Gain5/1  "uw_inv"
  Selector1/1 -> [is_uvw_pu_mod1]
  Gain/1 -> Bus Creator/4  "iu_inv_pu"
  Gain1/1 -> Bus Creator/5  "iv_inv_pu"
  Gain2/1 -> Bus Creator/6  "iw_inv_pu"
  Gain3/1 -> Bus Creator/1  "uu_inv_pu"
  Gain4/1 -> Bus Creator/2  "uv_inv_pu"
  Gain5/1 -> Bus Creator/3  "uw_inv_pu"
  connections:
  Current Sensor1/LConn1 -- Voltage Sensor1/LConn1 -- Voltage Sensor/RConn2 -- Uv/RConn1
  Voltage Sensor/RConn1 -- uu_inv/LConn1
  Current Sensor/RConn2 -- uu/RConn1
  Voltage Sensor1/RConn1 -- uv_inv/LConn1
  Voltage Sensor2/LConn1 -- Current Sensor2/LConn1 -- Voltage Sensor1/RConn2 -- Uw/RConn1
  Current Sensor/LConn1 -- Voltage Sensor2/RConn2 -- Uu/RConn1 -- Voltage Sensor/LConn1
  Current Sensor1/RConn2 -- uv/RConn1
  Voltage Sensor2/RConn1 -- uw_inv/LConn1
  iv_inv/LConn1 -- Current Sensor1/RConn1
  iu_inv/LConn1 -- Current Sensor/RConn1
  iw_inv/LConn1 -- Current Sensor2/RConn1
  Current Sensor2/RConn2 -- uw/RConn1

== system psm_sv_ekf_bemf_ctrl/inv_psm_mod1/inverter_ctrl/inverter_control/Speed control ==
  rotor speed : Inport
  rotor speed ref : Inport  Port=2
  1/Ti : Gain  Gain=kp_w  SaturateOnIntegerOverflow=on  OutDataTypeStr=Inherit: Same as input  ParamDataTypeStr=Inherit: Same as input
  Saturation : Saturate  UpperLimit=iq_lim  LowerLimit=-iq_lim
  Sum1 : Sum  Inputs=+++  SaturateOnIntegerOverflow=on
  Sum2 : Sum  Inputs=-+  SaturateOnIntegerOverflow=on
  Sum3 : Sum  Inputs=-+  SaturateOnIntegerOverflow=on
  Unit Delay4 : UnitDelay  SampleTime=-1
  kp : Gain  Gain=ki_w*ts_inv  SaturateOnIntegerOverflow=on  OutDataTypeStr=Inherit: Same as input  ParamDataTypeStr=Inherit: Same as input
  torque_ref : Outport
  wires:
  1/Ti/1 -> Sum1/1, Sum3/1
  kp/1 -> Sum1/2
  Sum3/1 -> Unit Delay4/1
  Unit Delay4/1 -> Sum1/3
  rotor speed ref/1 -> Sum2/2
  rotor speed/1 -> Sum2/1
  Sum2/1 -> kp/1, 1/Ti/1
  Sum1/1 -> Saturation/1
  Saturation/1 -> Sum3/2, torque_ref/1

== system psm_sv_ekf_bemf_ctrl/inv_psm_mod1/inverter_ctrl/inverter_control/current_ctrl ==
  torque_ref : Inport
  Bus Creator1 : BusCreator  Inputs=2
  EKF_bemf_observer : Subsystem
  current_ctrl : Subsystem
  current_transformation : Subsystem
  uab : Outport  VectorParamsAs1DForOutWhenUnconnected=off
  wires:
  [ubeta_pu_mod1] -> Bus Creator1/2  "ub"
  [ualpha_pu_mod1] -> Bus Creator1/1  "ua"
  Bus Creator1/1 -> uab/1
  torque_ref/1 -> current_ctrl/1(iq_ref)  "torque_ref"
  [ibeta_pu_mod1] -> EKF_bemf_observer/2(ibeta_pu)
  [ialpha_pu_mod1] -> EKF_bemf_observer/1(ialpha_pu)
  [ualpha_pu_mod1] -> EKF_bemf_observer/3(ualpha_pu)
  [ubeta_pu_mod1] -> EKF_bemf_observer/4(ubeta_pu)
  [udcd_pu_inv_mod1] -> current_ctrl/2(udc_pu), EKF_bemf_observer/5(udc_pu)

== system psm_sv_ekf_bemf_ctrl/inv_psm_mod1/inverter_ctrl/inverter_control/encoder-sensorless-switch ==
  MATLAB Function : MATLAB Function  TreatAsAtomicUnit=on
  Variant Source1 : VariantSource  VariantControls={use_psm_encoder == 1, use_psm_encoder == 0}
  Variant Source2 : VariantSource  VariantControls={use_psm_encoder == 1, use_psm_encoder == 0}
  double_integrator_observer : Subsystem
  omega_pu_psm/hat1 : Scope  NumInputPorts=2
      settings: ActiveDisplayYMinimum=-1  ActiveDisplayYMaximum=1  DataLoggingVariableName=ScopeData13
  phase_elec_psm/hat : Scope  NumInputPorts=2
      settings: ActiveDisplayYMinimum=-3.92695601880254  ActiveDisplayYMaximum=3.9266776333249296  DataLoggingVariableName=ScopeData12
  tag scope: motor_phase_ctrl_mod1=scoped, motor_speed_pu_ctrl_mod1=scoped
  wires:
  Variant Source1/1 -> [motor_speed_pu_ctrl_mod1]
  Variant Source2/1 -> [motor_phase_ctrl_mod1]
  [phase_hat_mod1] -> phase_elec_psm/hat/1  "theta_hat_mod1"
  [omega_hat_pu_mod1] -> omega_pu_psm/hat1/1  "omega_hat_pu_mod1"
  [phased_psm] -> double_integrator_observer/1(phase_psm)
  MATLAB Function/1(omega_ctrl) -> Variant Source1/2
  MATLAB Function/2(phase_ctrl) -> Variant Source2/2
  double_integrator_observer/1(phase_psm_hat) -> phase_elec_psm/hat/2, Variant Source2/1, MATLAB Function/1(phase_psm)  "phase_psm_hat"
  double_integrator_observer/2(omega_pu_psm_hat) -> Variant Source1/1, omega_pu_psm/hat1/2, MATLAB Function/2(omega_obs)  "omega_pu_psm_hat"
  [phase_hat_mod1] -> MATLAB Function/3(phase_obs)  "theta_hat_mod1"
  [omega_hat_pu_mod1] -> MATLAB Function/4(omega_psm)  "omega_hat_pu_mod1"

== system psm_sv_ekf_bemf_ctrl/inv_psm_mod1/inverter_ctrl/inverter_control/is inv quantizzation and one step delay ==
  is_abc_pu : Inport
  Demux : Demux  Outputs=3
  Mux : Mux  Inputs=3
  is inv quantizzation and one step delay : Subsystem
  isd_abc_pu : Outport
  wires:
  is inv quantizzation and one step delay/2(isd_v_pu) -> Mux/2
  is_abc_pu/1 -> Demux/1
  is inv quantizzation and one step delay/3(isd_w_pu) -> Mux/3
  is inv quantizzation and one step delay/1(isd_u_pu) -> Mux/1
  Demux/1 -> is inv quantizzation and one step delay/1(is_u_pu)
  Mux/1 -> isd_abc_pu/1
  Demux/3 -> is inv quantizzation and one step delay/3(is_w_pu)
  Demux/2 -> is inv quantizzation and one step delay/2(is_v_pu)

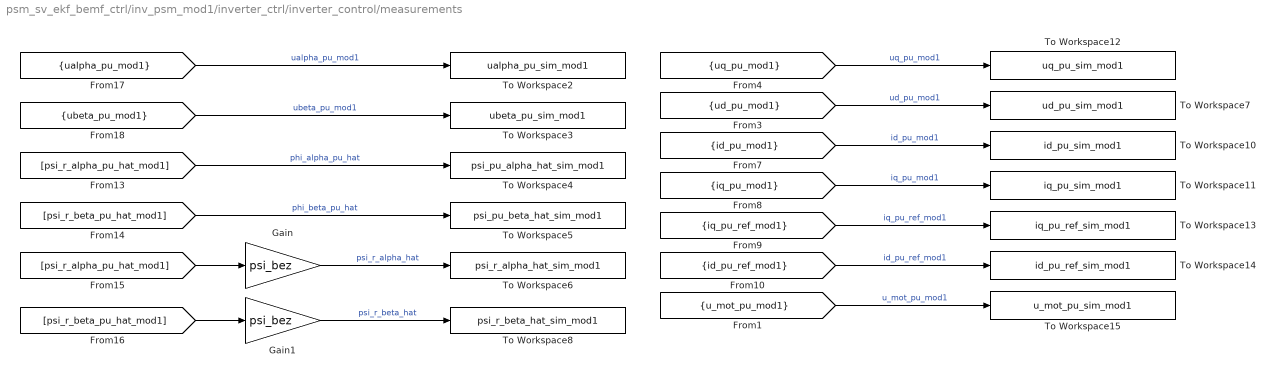
== system psm_sv_ekf_bemf_ctrl/inv_psm_mod1/inverter_ctrl/inverter_control/measurements ==
  Gain : Gain  Gain=psi_bez
  Gain1 : Gain  Gain=psi_bez
  To Workspace10 : ToWorkspace  VariableName=id_pu_sim_mod1  SampleTime=-1
      settings: MaxDataPoints=Ns_inv
  To Workspace11 : ToWorkspace  VariableName=iq_pu_sim_mod1  SampleTime=-1
      settings: MaxDataPoints=Ns_inv
  To Workspace12 : ToWorkspace  VariableName=uq_pu_sim_mod1  SampleTime=-1
      settings: MaxDataPoints=Ns_inv
  To Workspace13 : ToWorkspace  VariableName=iq_pu_ref_sim_mod1  SampleTime=-1
      settings: MaxDataPoints=Ns_inv
  To Workspace14 : ToWorkspace  VariableName=id_pu_ref_sim_mod1  SampleTime=-1
      settings: MaxDataPoints=Ns_inv
  To Workspace15 : ToWorkspace  VariableName=u_mot_pu_sim_mod1  SampleTime=-1
      settings: MaxDataPoints=Ns_inv
  To Workspace2 : ToWorkspace  VariableName=ualpha_pu_sim_mod1  SampleTime=-1
      settings: MaxDataPoints=Ns_inv
  To Workspace3 : ToWorkspace  VariableName=ubeta_pu_sim_mod1  SampleTime=-1
      settings: MaxDataPoints=Ns_inv
  To Workspace4 : ToWorkspace  VariableName=psi_pu_alpha_hat_sim_mod1  SampleTime=-1
      settings: MaxDataPoints=Ns_inv
  To Workspace5 : ToWorkspace  VariableName=psi_pu_beta_hat_sim_mod1  SampleTime=-1
      settings: MaxDataPoints=Ns_inv
  To Workspace6 : ToWorkspace  VariableName=psi_r_alpha_hat_sim_mod1  SampleTime=-1
      settings: MaxDataPoints=Ns_inv
  To Workspace7 : ToWorkspace  VariableName=ud_pu_sim_mod1  SampleTime=-1
      settings: MaxDataPoints=Ns_inv
  To Workspace8 : ToWorkspace  VariableName=psi_r_beta_hat_sim_mod1  SampleTime=-1
      settings: MaxDataPoints=Ns_inv
  wires:
  [psi_r_alpha_pu_hat_mod1] -> Gain/1
  [ualpha_pu_mod1] -> To Workspace2/1  "ualpha_pu_mod1"
  Gain/1 -> To Workspace6/1  "psi_r_alpha_hat"
  [psi_r_alpha_pu_hat_mod1] -> To Workspace4/1  "phi_alpha_pu_hat"
  [ubeta_pu_mod1] -> To Workspace3/1  "ubeta_pu_mod1"
  [psi_r_beta_pu_hat_mod1] -> To Workspace5/1  "phi_beta_pu_hat"
  Gain1/1 -> To Workspace8/1  "psi_r_beta_hat"
  [psi_r_beta_pu_hat_mod1] -> Gain1/1
  [u_mot_pu_mod1] -> To Workspace15/1  "u_mot_pu_mod1"
  [iq_pu_ref_mod1] -> To Workspace13/1  "iq_pu_ref_mod1"
  [ud_pu_mod1] -> To Workspace7/1  "ud_pu_mod1"
  [uq_pu_mod1] -> To Workspace12/1  "uq_pu_mod1"
  [iq_pu_mod1] -> To Workspace11/1  "iq_pu_mod1"
  [id_pu_mod1] -> To Workspace10/1  "id_pu_mod1"
  [id_pu_ref_mod1] -> To Workspace14/1  "id_pu_ref_mod1"

== system psm_sv_ekf_bemf_ctrl/inv_psm_mod1/inverter_ctrl/inverter_control/omega_acquisition ==
  omega_psm : Inport
  Gain : Gain  Gain=1/omega_bez
  Unit Delay : UnitDelay  SampleTime=-1
  Zero-Order Hold : ZeroOrderHold  SampleTime=-1
  omega_pu_psm : Outport
  wires:
  Zero-Order Hold/1 -> Gain/1
  omega_psm/1 -> Zero-Order Hold/1
  Unit Delay/1 -> omega_pu_psm/1
  Gain/1 -> Unit Delay/1

== system psm_sv_ekf_bemf_ctrl/inv_psm_mod1/inverter_ctrl/inverter_control/omega_pu ==
  Abs : Abs  SaturateOnIntegerOverflow=off
  flt : Subsystem
  abs(omega_pu) : Outport
  omega_pu : Outport  Port=2
  wires:
  Abs/1 -> flt/1(input)
  [motor_speed_pu_ctrl_mod1] -> Abs/1, omega_pu/1
  flt/1(output) -> abs(omega_pu)/1

== system psm_sv_ekf_bemf_ctrl/inv_psm_mod1/inverter_ctrl/inverter_control/phase_acquisition ==
  phase_psm : Inport
  Quantizer : Quantizer  QuantizationInterval=adc_quantization
  Unit Delay : UnitDelay  SampleTime=-1
  Zero-Order Hold : ZeroOrderHold  SampleTime=-1
  phased_psm : Outport
  wires:
  Zero-Order Hold/1 -> Quantizer/1
  Unit Delay/1 -> phased_psm/1
  phase_psm/1 -> Zero-Order Hold/1
  Quantizer/1 -> Unit Delay/1

== system psm_sv_ekf_bemf_ctrl/inv_psm_mod1/inverter_ctrl/inverter_control/phase_compensation_1 ==
  local_time : Inport
  master_time : Inport  Port=2
  Zero-Order Hold : ZeroOrderHold  SampleTime=-1
  Zero-Order Hold1 : ZeroOrderHold  SampleTime=-1
  alignment_ctrl : Subsystem
  y : Outport
  wires:
  local_time/1 -> Zero-Order Hold/1
  master_time/1 -> Zero-Order Hold1/1
  alignment_ctrl/1(dp) -> y/1
  Zero-Order Hold/1 -> alignment_ctrl/1(local_time)
  Zero-Order Hold1/1 -> alignment_ctrl/2(master_time)

== system psm_sv_ekf_bemf_ctrl/inv_psm_mod1/inverter_ctrl/inverter_control/speed_reference_generator ==
  Step : Step  Time=time_start_motor_control  FinalValue=omega_m_sim/omega_m_bez
  Step1 : Step  Commented=on  Time=simlength/2  FinalValue=-2*omega_m_sim/omega_m_bez
  Sum : Sum  Inputs=|++
  flt : Subsystem
  omega_ref_pu : Outport
  tag scope: omega_ref_pu_mod1=scoped
  wires:
  Step/1 -> Sum/1
  Step1/1 -> Sum/2
  Sum/1 -> flt/1(input)
  flt/1(output) -> [omega_ref_pu_mod1], omega_ref_pu/1

== system psm_sv_ekf_bemf_ctrl/inv_psm_mod1/inverter_ctrl/inverter_control/torque_reference ==
  rotor speed : Inport
  1-D Lookup Table : Lookup_n-D  NumberOfTableDimensions=1  BreakpointsForDimension1=rpm_base  Table=torque_base  InternalRulePriority=Speed  RndMeth=Simplest
  Gain : Gain  Gain=-1 %-1.45
  Gain1 : Gain  Gain=1/tau_bez
  Gain2 : Gain  Gain=rpm_bez
  Saturation : Saturate  UpperLimit=0  LowerLimit=-inf
  torque_ref : Outport
  wires:
  rotor speed/1 -> Gain2/1
  Saturation/1 -> torque_ref/1
  Gain1/1 -> Gain/1
  1-D Lookup Table/1 -> Gain1/1
  Gain2/1 -> 1-D Lookup Table/1
  Gain/1 -> Saturation/1

== system psm_sv_ekf_bemf_ctrl/inv_psm_mod1/inverter_ctrl/inverter_control/udc_acquisition ==
  udc_pu : Inport
  Quantizer : Quantizer  QuantizationInterval=adc_quantization
  Unit Delay : UnitDelay  SampleTime=-1
  Zero-Order Hold : ZeroOrderHold  SampleTime=-1
  udcd_pu : Outport
  wires:
  Quantizer/1 -> Unit Delay/1
  udc_pu/1 -> Zero-Order Hold/1
  Unit Delay/1 -> udcd_pu/1
  Zero-Order Hold/1 -> Quantizer/1
